simulink library "lib_DC_PES"  (R2026a)
settings: Solver=VariableStepAuto
undefined symbols (not defined in the file): block_buses, block_idx, block_toM, buses_lf, op_DC_PES
settings Model: Creator=atomas  LastModifiedBy=atomas

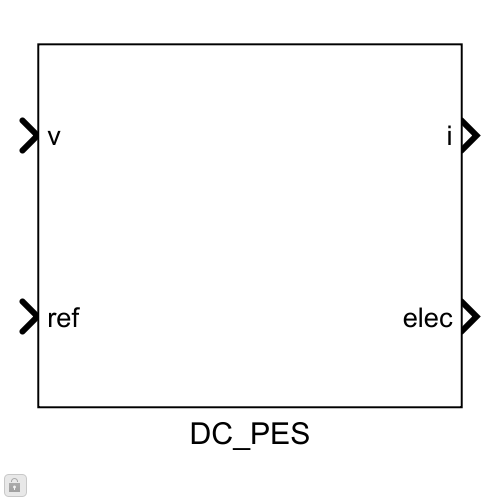
[thumbnail: Simulink's stored preview of the top-level diagram]
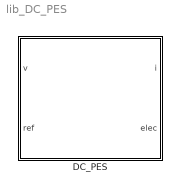
== system lib_DC_PES ==
  DC_PES : Subsystem  mask{Kp_dc=10, Ki_dc=10, T_pes=0.25, Kd_dc=0, T_wof=0.01}
      mask prompts: Kp_dc "DC-voltage proportional gain Kp_dc (pu):"; Ki_dc "DC-voltage integral gain Ki_dc (pu/s):"; T_pes "Primary energy source time constant T_pes (s):"; Kd_dc "DC-voltage derivative gain Kd_dc (pu*s):"; T_wof "Derivative washout time constant T_wof (s):"
      mask init:
      | [block_buses, block_Pg, block_toM, block_idx, use_wof] = mask_init_DC_PES(gcb, Kd_dc);

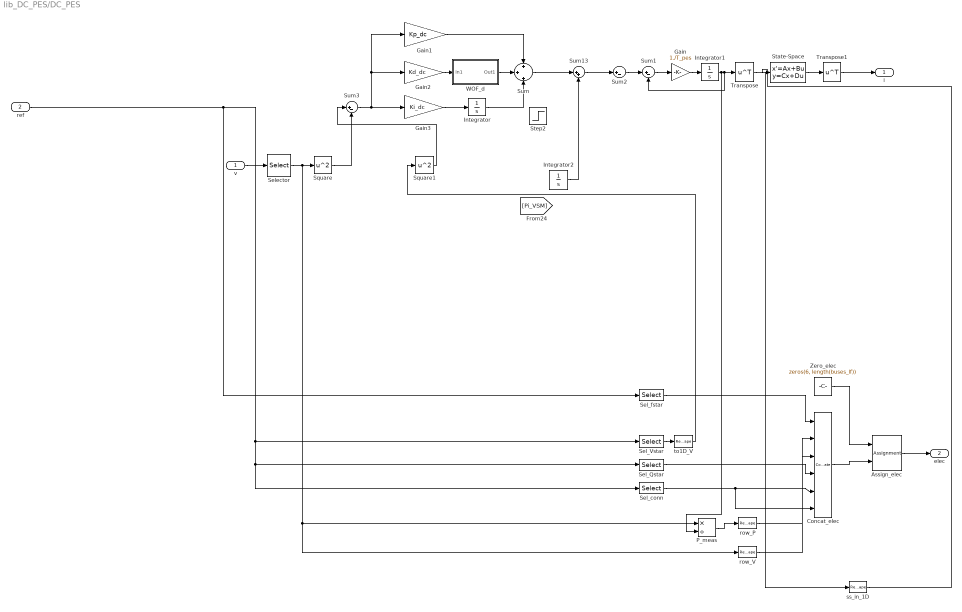
== system lib_DC_PES/DC_PES ==
  v : Inport
  ref : Inport  Port=2
  Assign_elec : Assignment  NumberOfDimensions=2  DiagnosticForDimensions=Warning  IndexOptions=Assign all,Index vector (dialog)  Indices=1,block_idx  OutputSizes=1
  Concat_elec : Concatenate  NumInputs=6  Mode=Multidimensional array
  Gain : Gain  Gain=1./T_pes
  Gain1 : Gain  Gain=Kp_dc
  Gain2 : Gain  Gain=Kd_dc
  Gain3 : Gain  Gain=Ki_dc
  Integrator : Integrator  InitialCondition=op_DC_PES.Integrator
  Integrator1 : Integrator  InitialCondition=op_DC_PES.Integrator1
  Integrator2 : Integrator  InitialCondition=op_DC_PES.Integrator2
  P_meas : Product  Inputs=*/
  Sel_Qstar : Selector  NumberOfDimensions=2  InputPortWidth=3  IndexOptions=Index vector (dialog),Index vector (dialog)  Indices=4,block_idx  OutputSizes=1
  Sel_Vstar : Selector  NumberOfDimensions=2  InputPortWidth=3  IndexOptions=Index vector (dialog),Index vector (dialog)  Indices=3,block_idx  OutputSizes=1
  Sel_conn : Selector  NumberOfDimensions=2  InputPortWidth=3  IndexOptions=Index vector (dialog),Index vector (dialog)  Indices=5,block_idx  OutputSizes=1
  Sel_fstar : Selector  NumberOfDimensions=2  InputPortWidth=3  IndexOptions=Index vector (dialog),Index vector (dialog)  Indices=1,block_idx  OutputSizes=1
  Selector : Selector  InputPortWidth=DC.Nbuses  IndexOptions=Index vector (dialog)  Indices=block_buses  OutputSizes=1
  Square : Math  Operator=square
  Square1 : Math  Operator=square
  State-Space : StateSpace  A=[]  B=[]  C=[]  D=block_toM  InitialCondition=0  ParameterTunability=Optimized
  Step2 : Step  Time=0.1  FinalValue=0.1  SampleTime=0
  Sum : Sum  Inputs=+|+|+
  Sum1 : Sum  Inputs=|+-
  Sum13 : Sum  Inputs=|++
  Sum2 : Sum  Inputs=|+-
  Sum3 : Sum  Inputs=|+-
  Transpose : Math  Operator=transpose
  Transpose1 : Math  Operator=transpose
  WOF_d : Subsystem  Variant=on
  Zero_elec : Constant  Value=zeros(6, length(buses_lf))
  row_P : Reshape  OutputDimensionality=Customize  OutputDimensions=[1, length(block_buses)]
  row_V : Reshape  OutputDimensionality=Customize  OutputDimensions=[1, length(block_buses)]
  ss_in_1D : Reshape
  to1D_V : Reshape
  i : Outport
  elec : Outport  Port=2
  wires:
  WOF_d/1(Out1) -> Sum/2
  Gain2/1 -> WOF_d/1(In1)
  State-Space/1 -> Transpose1/1
  Transpose1/1 -> i/1
  Sum3/1 -> Gain2/1, Gain1/1, Gain3/1
  v/1 -> Selector/1
  Selector/1 -> P_meas/1, row_V/1, Square/1
  Sum1/1 -> Gain/1
  Integrator1/1 -> Sum1/2, Transpose/1, P_meas/2
  Gain/1 -> Integrator1/1
  Sum2/1 -> Sum1/1
  Sum13/1 -> Sum2/1
  Integrator2/1 -> Sum13/2
  Sum/1 -> Sum13/1
  Gain3/1 -> Integrator/1
  Square/1 -> Sum3/2
  Gain1/1 -> Sum/1
  Integrator/1 -> Sum/3
  ref/1 -> Sel_Qstar/1, Sel_conn/1, Sel_Vstar/1, Sel_fstar/1
  Sel_fstar/1 -> Concat_elec/1
  Sel_Qstar/1 -> Concat_elec/4
  Sel_conn/1 -> Concat_elec/5, Concat_elec/6
  Zero_elec/1 -> Assign_elec/1
  Concat_elec/1 -> Assign_elec/2
  Assign_elec/1 -> elec/1
  Sel_Vstar/1 -> to1D_V/1
  P_meas/1 -> row_P/1
  row_P/1 -> Concat_elec/2
  row_V/1 -> Concat_elec/3
  Transpose/1 -> ss_in_1D/1
  ss_in_1D/1 -> State-Space/1
  to1D_V/1 -> Square1/1
  Square1/1 -> Sum3/1

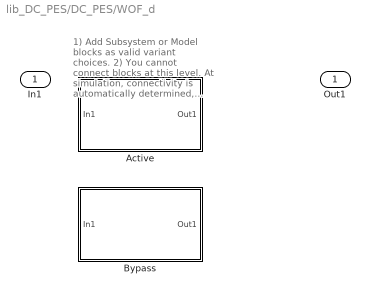
== system lib_DC_PES/DC_PES/WOF_d ==
  note: 1) Add Subsystem or Model blocks as valid variant choices.
      | 2) You cannot connect blocks at this level. At simulation, connectivity is automatically
      | determined, based on the active variant and port name matching.
  In1 : Inport
  Active : Subsystem  VariantControl=use_wof == 1
  Bypass : Subsystem  VariantControl=(default)
  Out1 : Outport

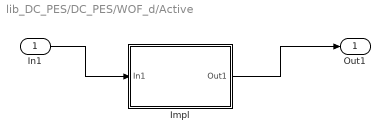
== system lib_DC_PES/DC_PES/WOF_d/Active ==
  In1 : Inport
  Impl : Subsystem
  Out1 : Outport
  wires:
  Impl/1(Out1) -> Out1/1
  In1/1 -> Impl/1(In1)

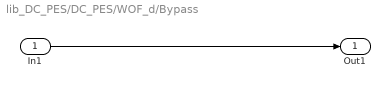
== system lib_DC_PES/DC_PES/WOF_d/Bypass ==
  In1 : Inport
  Out1 : Outport
  wires:
  In1/1 -> Out1/1

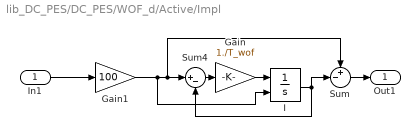
== system lib_DC_PES/DC_PES/WOF_d/Active/Impl ==
  In1 : Inport
  Gain : Gain  Gain=1./T_wof
  Gain1 : Gain  Gain=100
  I : Integrator  InitialConditionSource=external  InitialCondition=op_DC_PES.WOF_d_Active_Impl_I
  Sum : Sum  Inputs=+-|
  Sum4 : Sum  Inputs=|+-
  Out1 : Outport
  wires:
  Gain1/1 -> Sum/1, Sum4/1, I/2
  Gain/1 -> I/1
  Sum4/1 -> Gain/1
  In1/1 -> Gain1/1
  I/1 -> Sum/2, Sum4/2
  Sum/1 -> Out1/1
